simulink model "QD2_DroneStack_MPC"  (R2025a)
settings: Solver=ode1  StartTime=0.0  StopTime=inf  FixedStep=1/1000  RelTol=1e-3  EnableMultiTasking=on
InitFcn:
  | % QD2_DroneStack_MPC: rutas de la librería qd2_* y del mapeo de motores
  | qd2_d = fileparts(get_param(bdroot, 'FileName'));
  | for qd2_k = 1:4
  |     if exist(fullfile(qd2_d, 'lib', 'qd2_params.m'), 'file'), break; end
  |     qd2_d = fileparts(qd2_d);
  | end
  | addpath(fullfile(qd2_d, 'lib'));
  | addpath(fullfile(qd2_d, 'equipo2_original'));
  | clear qd2_d qd2_k
  | Motor_Mapping_7_Inch
model workspace (MAT data in the model file):
  target_system = 1
undefined symbols (not defined in the file): _Commander, _QDrone2, _Stabilizer, datetime, HIL, KT, lf, log_, m, Motor_Matrix, n, qc_get_step_size, s, saved_data
libraries: quarc_library x94, simulink x27, simulink_extras x9
(part 5 of 5)

== matlab function QD2_DroneStack_MPC/QDrone2 DAQ/MotorCMD_FSM ==
  data: Arm_Signal input; E_Stop input; ESC_cmd output; Motor_State output; Model_Time input; Motor_State input
function [ESC_cmd,Motor_State]= fcn(Arm_Signal,E_Stop,Model_Time, Motor_State)

persistent state ESC_CMD 

%  Initialize motor state at the start of the model
if isempty(state)
    state = 2;
    ESC_CMD = zeros(1,4);
end 

% ESC Numbers w.r.t motor positions on QDrone: 
%         FRONT
%       4(3)       2(1)
% 
%       3(2)       1(0)
%          BACK  


% ============ Motor programing state machine ============ 

% State machine transitions: 

% Motor configuration state: 
if E_Stop == 0 && state ~= 9
    % Start with the motors in an idle state    
    if state == 2 && Model_Time > 0 && Model_Time <= 1  
        if Arm_Signal == 1
            % Error state, you started the model while the QDrone was armed
            state = 9;
        end 
           
    elseif state ==2  && Model_Time > 1 && Model_Time <= 2
        % Enter motor Low Frequency state:
        state = 1;
        
    elseif state ==1  && Model_Time > 2 && Model_Time <= 2.5
        % Set motor orientation
        state = 0;
        
    elseif state == 0 && Model_Time > 2.5    
        % Enter motor idle state: 
        state = 2; 

    elseif Motor_State ==2 && Arm_Signal == 1 
        % Enter arm state 
        state = 3;

    elseif Motor_State ==3 && Arm_Signal ==0 
        % Return to idle state 
        state = 2; 
    end 
    
elseif E_Stop ==1 
    % You've entered emergency state, disarm QDrone2!
    state = 9; 
end 


% State Machine commands: 
switch state 
    
    % ESC orientation set:
    case 0
        % for all drones
        ESC_CMD = [20,21,21,20];
        %for 1st R&D Drone 
        % ESC_CMD = [0,0,0,0];
    
    % Motor Low Frequency Beep:
    case 1
        ESC_CMD = [1,1,1,1];
    
    % Enter motor stop state: 
    case 2
        ESC_CMD = [0,0,0,0];
    
    % Motors in Arm State:
    case 3
        ESC_CMD = [48,48,48,48];
        
    % Same as state 2 but used as an Error State to stop motor cmd:
    case 9
        ESC_CMD = [0,0,0,0];
        
end 
    


Motor_State = state;
ESC_cmd = ESC_CMD;

Motor_State, ESC_cmd;

== matlab function QD2_DroneStack_MPC/HORIZON FRAME CONVERSION AND ESTIMATION/Pose Switchbox/MATLAB Function ==
  data: sigmoid_type input; enable output; x_des input; slow_lim input; fast_lim input; x_cur input; x_vel input; x_ref output; max_x_vel output; max_x_accel output; x_meas input
function [enable, x_ref, max_x_vel, max_x_accel] = fcn(sigmoid_type, x_des, slow_lim, fast_lim, x_cur, x_vel, x_meas)

% Note: Some of the cases below are identical. However, they are separated out 
% based on the states of the state machine for ease of modification in the future. 
% For example, states 4 and 5 are identical. However, if the user wants different 
% signmoid behaviour when taking off than when landing, these cases may not be the same. 

enable = 0;
x_ref = 0;
max_x_vel = 0;
max_x_accel = 0;

switch sigmoid_type
    case 1 % This is for the IDLE, ARM, E_ABORT, E_STOP and DISABLE states of the FSM
        enable = 1;
        x_ref = x_meas;
        max_x_vel = slow_lim(1);
        max_x_accel = slow_lim(2);

    case 2 % This is for the TAKEOFF THROTTLE state of the FSM
        enable = 1;
        x_ref = x_meas;
        max_x_vel = slow_lim(1);
        max_x_accel = slow_lim(2);

    case 3 % This is for the FLIGHT state of the FSM
        enable = 1;
        x_ref = x_des;
        max_x_vel = fast_lim(1);
        max_x_accel = fast_lim(2);

    case 4 % This is for the TAKEOFF HEIGHT state of the FSM
        enable = 1;
        x_ref = x_des;
        if (abs(x_cur - x_des) <= 0.02)
            max_x_vel = fast_lim(1);
            max_x_accel = fast_lim(2);
        else    
            max_x_vel = slow_lim(1);
            max_x_accel = slow_lim(2);
        end
    case 5 % This is for the AUTOLAND state of the FSM
        enable = 1;
        x_ref = x_des;
        if (abs(x_cur - x_des) <= 0.02)
            max_x_vel = fast_lim(1);
            max_x_accel = fast_lim(2);        
        else
            max_x_vel = slow_lim(1);
            max_x_accel = slow_lim(2);
        end
        
end

== matlab function QD2_DroneStack_MPC/HORIZON FRAME CONVERSION AND ESTIMATION/Pose Switchbox/MATLAB Function1 ==
  data: sigmoid_type input; enable output; y_des input; slow_lim input; fast_lim input; y_cur input; y_vel input; y_ref output; max_y_vel output; max_y_accel output; y_meas input
function [enable, y_ref, max_y_vel, max_y_accel] = fcn(sigmoid_type, y_des, slow_lim, fast_lim, y_cur, y_vel, y_meas)

% Note: Some of the cases below are identical. However, they are separated out 
% based on the states of the state machine for ease of modification in the future. 
% For example, states 4 and 5 are identical. However, if the user wants different 
% signmoid behaviour when taking off than when landing, these cases may not be the same. 

enable = 0;
y_ref = 0;
max_y_vel = 0;
max_y_accel = 0;

switch sigmoid_type
    case 1 % This is for the IDLE, ARM, E_ABORT, E_STOP and DISABLE states of the FSM
        enable = 1;
        y_ref = y_meas;
        max_y_vel = slow_lim(1);
        max_y_accel = slow_lim(2);

    case 2 % This is for the TAKEOFF THROTTLE state of the FSM
        enable = 1;
        y_ref = y_meas;
        max_y_vel = slow_lim(1);
        max_y_accel = slow_lim(2);

    case 3 % This is for the FLIGHT state of the FSM
        enable = 1;
        y_ref = y_des;
        max_y_vel = fast_lim(1);
        max_y_accel = fast_lim(2);

    case 4 % This is for the TAKEOFF HEIGHT state of the FSM
        enable = 1;
        y_ref = y_des;
        if (abs(y_cur - y_des) <= 0.02)
            max_y_vel = fast_lim(1);
            max_y_accel = fast_lim(2);
        else    
            max_y_vel = slow_lim(1);
            max_y_accel = slow_lim(2);
        end
    case 5 % This is for the AUTOLAND state of the FSM
        enable = 1;
        y_ref = y_des;
        if (abs(y_cur - y_des) <= 0.02)
            max_y_vel = fast_lim(1);
            max_y_accel = fast_lim(2);        
        else
            max_y_vel = slow_lim(1);
            max_y_accel = slow_lim(2);
        end
        
end
